simulink library "GridPackLib2"  (R2025b)
settings: Solver=VariableStepAuto  StartTime=0.0  StopTime=10.0  RelTol=1e-3
undefined symbols (not defined in the file): battery_builder_rtmsupport, gcbh
libraries: GridPackLib2_lib x2, nesl_utility x2
settings Model: Creator=User  LastModifiedBy=User

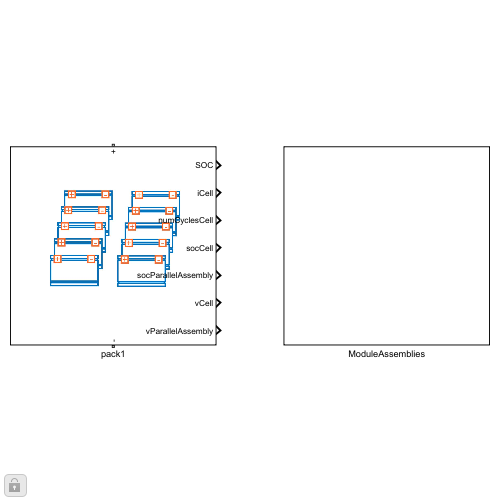
[thumbnail: Simulink's stored preview of the top-level diagram]
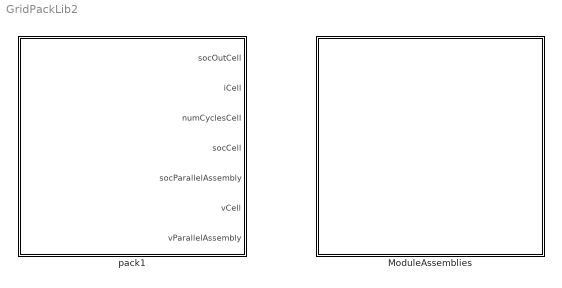
== system GridPackLib2 ==
  ModuleAssemblies : Subsystem
  pack1 : Subsystem  LoadFcn=battery_builder_rtmsupport('loadfcn',gcbh);
      settings: CopyFcn=battery_builder_rtmsupport('copyfcn',gcbh);  PreCopyFcn=battery_builder_rtmsupport('precopyfcn',gcbh);  PreDeleteFcn=battery_builder_rtmsupport('predeletefcn',gcbh);  PortSchema="{\"entries\":[{\"content\":{\"sides\":[{\"content\":{\"connectorIds\":[\"LConn1\"]},\"type\":\"ConnectorPlacement.EquallySpacedRectSide\",\"uuid\":\"88f5d390-8915-47fe-8d71-24cfaf6a6e27\"},{\"content\":{\"connectorIds\":[\"RConn1\"],\"side\":\"RIGHT\"},\"type\":\"ConnectorPlacement.EquallySpacedRectSide\",\"uuid\":\"89ebc1e9-5c7a-4e3e-b4ce-2bf86473cd1d\"},{\"content\":{\"side\":\"TOP\"},\"type\":\"ConnectorPlacement.EquallySpacedRectSide\",\"uuid\":\"3176116c-a81f-42a8-8903-646dc7856346\"},{\"content\":{\"connectorIds\":[\"Out1\",\"Out2\",\"Out3\",\"Out4\",\"Out5\",\"Out6\",\"Out7\"],\"side\":\"BOTTOM\"},\"type\":\"ConnectorPlacement.EquallySpacedRectSide\",\"uuid\":\"28216ba3-1a22-4e70-aa06-090b301a362d\"}]},\"type\":\"ConnectorPlacement.EquallySpacedConnector\",\"uuid\":\"25e0ce26-fb40-4ff1-8f8a-65e5050e8f25\"}],\"packageUris\":[\"http://schema.mathworks.com/mf0/Connector/R2020b\"],\"version\":\"1.0\"}"
      mask Display: image('$imagefile')

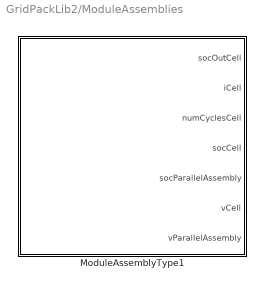
== system GridPackLib2/ModuleAssemblies ==
  ModuleAssemblyType1 : Subsystem  LoadFcn=battery_builder_rtmsupport('loadfcn',gcbh);
      settings: CopyFcn=battery_builder_rtmsupport('copyfcn',gcbh);  PreCopyFcn=battery_builder_rtmsupport('precopyfcn',gcbh);  PreDeleteFcn=battery_builder_rtmsupport('predeletefcn',gcbh);  PortSchema="{\"entries\":[{\"content\":{\"sides\":[{\"content\":{\"connectorIds\":[\"LConn1\"]},\"type\":\"ConnectorPlacement.EquallySpacedRectSide\",\"uuid\":\"88f5d390-8915-47fe-8d71-24cfaf6a6e27\"},{\"content\":{\"connectorIds\":[\"RConn1\"],\"side\":\"RIGHT\"},\"type\":\"ConnectorPlacement.EquallySpacedRectSide\",\"uuid\":\"89ebc1e9-5c7a-4e3e-b4ce-2bf86473cd1d\"},{\"content\":{\"side\":\"TOP\"},\"type\":\"ConnectorPlacement.EquallySpacedRectSide\",\"uuid\":\"3176116c-a81f-42a8-8903-646dc7856346\"},{\"content\":{\"connectorIds\":[\"Out1\",\"Out2\",\"Out3\",\"Out4\",\"Out5\",\"Out6\",\"Out7\"],\"side\":\"BOTTOM\"},\"type\":\"ConnectorPlacement.EquallySpacedRectSide\",\"uuid\":\"a9e7f8c6-f04c-4c1e-b058-680dc39e5ef0\"}]},\"type\":\"ConnectorPlacement.EquallySpacedConnector\",\"uuid\":\"25e0ce26-fb40-4ff1-8f8a-65e5050e8f25\"}],\"packageUris\":[\"http://schema.mathworks.com/mf0/Connector/R2020b\"],\"version\":\"1.0\"}"
      mask Display: image('$imagefile')

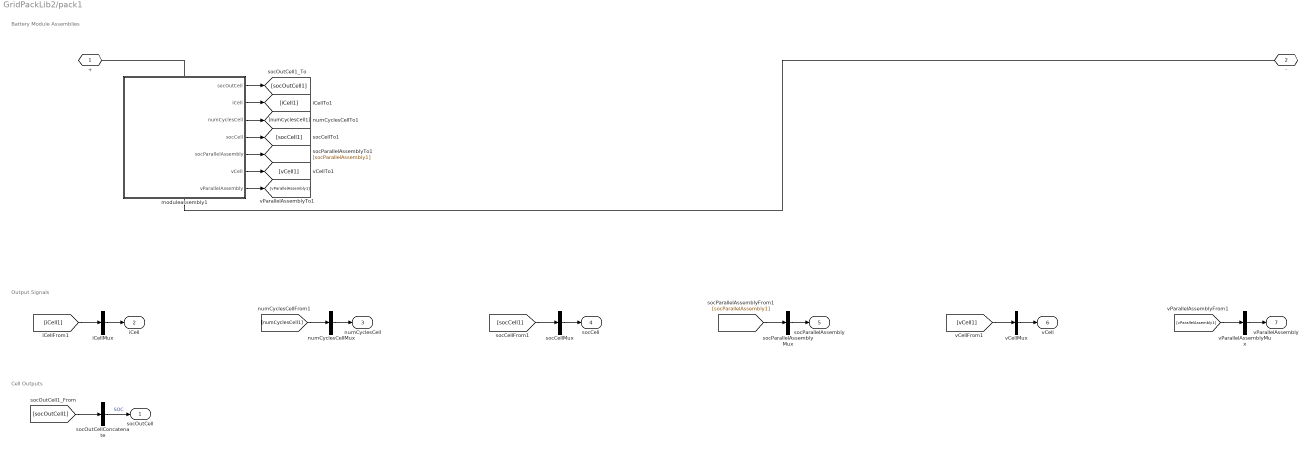
== system GridPackLib2/pack1 ==
  note: Battery Module Assemblies
  note: Output Signals
  note: Cell Outputs
  iCellMux : Mux  Inputs=1
  moduleassembly1 : Subsystem  LoadFcn=battery_builder_rtmsupport('loadfcn',gcbh);
      settings: CopyFcn=battery_builder_rtmsupport('copyfcn',gcbh);  PreCopyFcn=battery_builder_rtmsupport('precopyfcn',gcbh);  PreDeleteFcn=battery_builder_rtmsupport('predeletefcn',gcbh);  PortSchema="{\"entries\":[{\"content\":{\"sides\":[{\"content\":{\"connectorIds\":[\"LConn1\"]},\"type\":\"ConnectorPlacement.EquallySpacedRectSide\",\"uuid\":\"88f5d390-8915-47fe-8d71-24cfaf6a6e27\"},{\"content\":{\"connectorIds\":[\"RConn1\"],\"side\":\"RIGHT\"},\"type\":\"ConnectorPlacement.EquallySpacedRectSide\",\"uuid\":\"89ebc1e9-5c7a-4e3e-b4ce-2bf86473cd1d\"},{\"content\":{\"side\":\"TOP\"},\"type\":\"ConnectorPlacement.EquallySpacedRectSide\",\"uuid\":\"3176116c-a81f-42a8-8903-646dc7856346\"},{\"content\":{\"connectorIds\":[\"Out1\",\"Out2\",\"Out3\",\"Out4\",\"Out5\",\"Out6\",\"Out7\"],\"side\":\"BOTTOM\"},\"type\":\"ConnectorPlacement.EquallySpacedRectSide\",\"uuid\":\"a9e7f8c6-f04c-4c1e-b058-680dc39e5ef0\"}]},\"type\":\"ConnectorPlacement.EquallySpacedConnector\",\"uuid\":\"25e0ce26-fb40-4ff1-8f8a-65e5050e8f25\"}],\"packageUris\":[\"http://schema.mathworks.com/mf0/Connector/R2020b\"],\"version\":\"1.0\"}"
      mask Display: image('$imagefile')
  numCyclesCellMux : Mux  Inputs=1
  socCellMux : Mux  Inputs=1
  socOutCellConcatenate : Concatenate  NumInputs=1  Mode=Multidimensional array  ConcatenateDimension=2
  socParallelAssemblyMux : Mux  Inputs=1
  vCellMux : Mux  Inputs=1
  vParallelAssemblyMux : Mux  Inputs=1
  + : PMIOPort  Side=Left
  - : PMIOPort  Port=2  Side=Right
  socOutCell : Outport
  iCell : Outport  Port=2
  numCyclesCell : Outport  Port=3
  socCell : Outport  Port=4
  socParallelAssembly : Outport  Port=5
  vCell : Outport  Port=6
  vParallelAssembly : Outport  Port=7
  wires:
  socOutCellConcatenate/1 -> socOutCell/1  "SOC"
  [socOutCell1] -> socOutCellConcatenate/1
  moduleassembly1/2(iCell) -> [iCell1]
  iCellMux/1 -> iCell/1
  [iCell1] -> iCellMux/1
  moduleassembly1/3(numCyclesCell) -> [numCyclesCell1]
  numCyclesCellMux/1 -> numCyclesCell/1
  [numCyclesCell1] -> numCyclesCellMux/1
  moduleassembly1/4(socCell) -> [socCell1]
  socCellMux/1 -> socCell/1
  [socCell1] -> socCellMux/1
  moduleassembly1/5(socParallelAssembly) -> [socParallelAssembly1]
  socParallelAssemblyMux/1 -> socParallelAssembly/1
  [socParallelAssembly1] -> socParallelAssemblyMux/1
  moduleassembly1/6(vCell) -> [vCell1]
  vCellMux/1 -> vCell/1
  [vCell1] -> vCellMux/1
  moduleassembly1/7(vParallelAssembly) -> [vParallelAssembly1]
  vParallelAssemblyMux/1 -> vParallelAssembly/1
  [vParallelAssembly1] -> vParallelAssemblyMux/1
  moduleassembly1/1(socOutCell) -> [socOutCell1]
  connections:
  moduleassembly1/LConn1 -- +/RConn1
  moduleassembly1/RConn1 -- -/RConn1

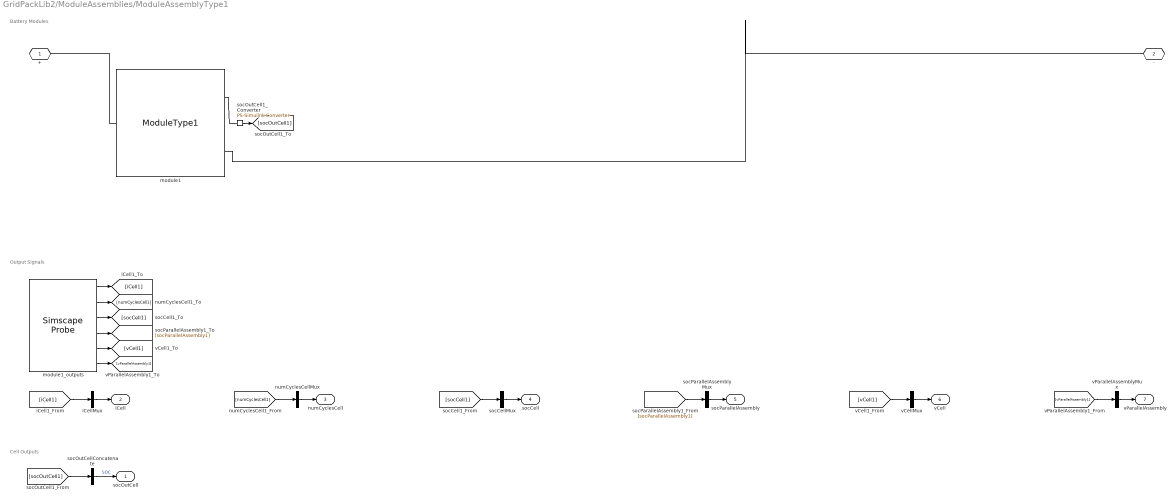
== system GridPackLib2/ModuleAssemblies/ModuleAssemblyType1 ==
  note: Battery Modules
  note: Output Signals
  note: Cell Outputs
  iCellMux : Mux  Inputs=1
  module1 : GridPackLib2_lib/Modules/ModuleType1  SOC_vecCell=[0, .01, .02, .03, .04, .05, .06, .07, .08, .09, .1, .11, .12, .13, .14, .15, .16, .17, .18, .19, .2, .21, .22, .23, .24, .25, .26, .27, .28, .29, .3, .31, .32, .33, .34, .35, .36, .37, .38, .39, .4, .41, .42, .43, .44, .45, .46, .47, .48, .49, .5, .51, .52, .53, .54, .55, .56, .57, .58, .59, .6, .61, .62, .63, .64, .65, .66, .67, .68, .69, .7, .71, .72, .73, .74, .75, .76, .77, .78, .79, .8, .81, .82, .83, .84, .85, .86, .87, .88, .89, .9, .91, .92, .93, .94, .95, .96, .97, .98, .99, 1]  V0_vecCell=[2.74087, 2.86425, 2.94379, 3.04526, 3.12652, 3.19558, 3.2527, 3.29775, 3.33159, 3.36, 3.3837, 3.4034, 3.41925, 3.43509, 3.4486, 3.45932, 3.47006, 3.47863, 3.48489, 3.49188, 3.49842, 3.50409, 3.50964, 3.51584, 3.52204, 3.52785, 3.53338, 3.53848, 3.54356, 3.54863, 3.55351, 3.55882, 3.56372, 3.56861, 3.5735, 3.57836, 3.58329, 3.58821, 3.59317, 3.59804, 3.60332, 3.60907, 3.61483, 3.62059, 3.62652, 3.6327, 3.63888, 3.64585, 3.65366, 3.66147, 3.66917, 3.67655, 3.68392, 3.69145, 3.69898, 3.70781, 3.71738, 3.72696, 3.73653, 3.74624, 3.75595, 3.7653, 3.77428, 3.7832, 3.79205, 3.8007, 3.80927, 3.8178, 3.82625, 3.83464, 3.84361, 3.85255, 3.86146, 3.87037, 3.87823, 3.88606, 3.89449, 3.90374, 3.91298, 3.9226, 3.93231, 3.94199, 3.95307, 3.96471, 3.97635, 3.98832, 4.00042, 4.01239, 4.02377, 4.03506, 4.04653, 4.05796, 4.06839, 4.07872, 4.08848, 4.09766, 4.10666, 4.11624, 4.12852, 4.14359, 4.22965] V  V_rangeCell=[2.475, Inf] V  R0_vecCell=[.3952, .44824, .45817, .49649, .51801, .52941, .53219, .52804, .51966, .50893, .49666, .48177, .46682, .45187, .43666, .42292, .40923, .39435, .37836, .3654, .35267, .33913, .32835, .31969, .31103, .30202, .29449, .28761, .28074, .27387, .26782, .26352, .25908, .25465, .2502, .2454, .24066, .23593, .23117, .22626, .22256, .22016, .21777, .21537, .21336, .21163, .20989, .20874, .20837, .208, .20731, .20564, .20397, .20226, .20055, .20026, .20086, .20147, .20207, .20264, .2032, .20269, .20183, .20093, .20005, .19903, .19783, .19654, .19527, .19397, .19325, .19243, .19151, .1906, .1887, .18671, .18502, .18504, .18507, .18543, .18518, .18483, .18547, .18641, .18735, .18945, .19195, .19411, .19486, .19553, .19661, .19791, .19879, .19998, .20083, .20074, .1989, .19723, .19215, .18252, .02326] Ohm  AHCell=0.716 A*hr  extrapolation_optionCell=simscape.enum.extrapolation.nearest  P=44  S=100  iCell_specify=off  iCell_priority=None  iCell=0 A  iCell_nominal_specify=off  iCell_nominal_value=1  iCell_nominal_unit=A  vCell_specify=off  vCell_priority=None  vCell=0 V  vCell_nominal_specify=off  vCell_nominal_value=1  vCell_nominal_unit=V  socCell_specify=off  socCell_priority=High  socCell=1  socCell_nominal_specify=off  socCell_nominal_value=1  socCell_nominal_unit=1  numCyclesCell_specify=off  numCyclesCell_priority=High  numCyclesCell=0  numCyclesCell_nominal_specify=off  numCyclesCell_nominal_value=1  numCyclesCell_nominal_unit=1  vParallelAssembly_specify=off  vParallelAssembly_priority=None  vParallelAssembly=repmat(0, 100, 1) V  vParallelAssembly_nominal_specify=off  vParallelAssembly_nominal_value=1  vParallelAssembly_nominal_unit=V  socParallelAssembly_specify=off  socParallelAssembly_priority=None  socParallelAssembly=repmat(1, 100, 1)  socParallelAssembly_nominal_specify=off  socParallelAssembly_nominal_value=1  socParallelAssembly_nominal_unit=1
      settings: InternalSimscapePortConfiguration="{\"Bottom\":[{\"id\":\"n\",\"label\":\"-\",\"type\":\"foundation.electrical.electrical\"}],\"Left\":[],\"Right\":[{\"id\":\"socOutCell\",\"label\":\"SOC\",\"type\":\"output\"}],\"Top\":[{\"id\":\"p\",\"label\":\"+\",\"type\":\"foundation.electrical.electrical\"}]}"
  module1_outputs : SimscapeProbe  BoundBlock=3  Variables="{\"iCell\":{\"Probing\":\"ON\"},\"numCyclesCell\":{\"Probing\":\"ON\"},\"socCell\":{\"Probing\":\"ON\"},\"socParallelAssembly\":{\"Probing\":\"ON\"},\"vCell\":{\"Probing\":\"ON\"},\"vParallelAssembly\":{\"Probing\":\"ON\"}}"
  numCyclesCellMux : Mux  Inputs=1
  socCellMux : Mux  Inputs=1
  socOutCell1_Converter : nesl_utility/PS-Simulink Converter  PhysicalDomain=network_engine_domain  SubClassName=ps_output  LeftPortType=input  RightPortType=output  PseudoPeriodic=off  Frequencies=[]  VectorFormat=inherit  Unit=inherit  AffineConversion=off
  socOutCellConcatenate : Concatenate  NumInputs=1  Mode=Multidimensional array  ConcatenateDimension=2
  socParallelAssemblyMux : Mux  Inputs=1
  vCellMux : Mux  Inputs=1
  vParallelAssemblyMux : Mux  Inputs=1
  + : PMIOPort  Side=Left
  - : PMIOPort  Port=2  Side=Right
  socOutCell : Outport
  iCell : Outport  Port=2
  numCyclesCell : Outport  Port=3
  socCell : Outport  Port=4
  socParallelAssembly : Outport  Port=5
  vCell : Outport  Port=6
  vParallelAssembly : Outport  Port=7
  wires:
  socOutCellConcatenate/1 -> socOutCell/1  "SOC"
  [socOutCell1] -> socOutCellConcatenate/1
  module1_outputs/1 -> [iCell1]
  iCellMux/1 -> iCell/1
  [iCell1] -> iCellMux/1
  module1_outputs/2 -> [numCyclesCell1]
  numCyclesCellMux/1 -> numCyclesCell/1
  [numCyclesCell1] -> numCyclesCellMux/1
  module1_outputs/3 -> [socCell1]
  socCellMux/1 -> socCell/1
  [socCell1] -> socCellMux/1
  module1_outputs/4 -> [socParallelAssembly1]
  socParallelAssemblyMux/1 -> socParallelAssembly/1
  [socParallelAssembly1] -> socParallelAssemblyMux/1
  module1_outputs/5 -> [vCell1]
  vCellMux/1 -> vCell/1
  [vCell1] -> vCellMux/1
  module1_outputs/6 -> [vParallelAssembly1]
  vParallelAssemblyMux/1 -> vParallelAssembly/1
  [vParallelAssembly1] -> vParallelAssemblyMux/1
  socOutCell1_Converter/1 -> [socOutCell1]
  connections:
  module1/LConn1 -- +/RConn1
  module1/RConn2 -- -/RConn1
  socOutCell1_Converter/LConn1 -- module1/RConn1

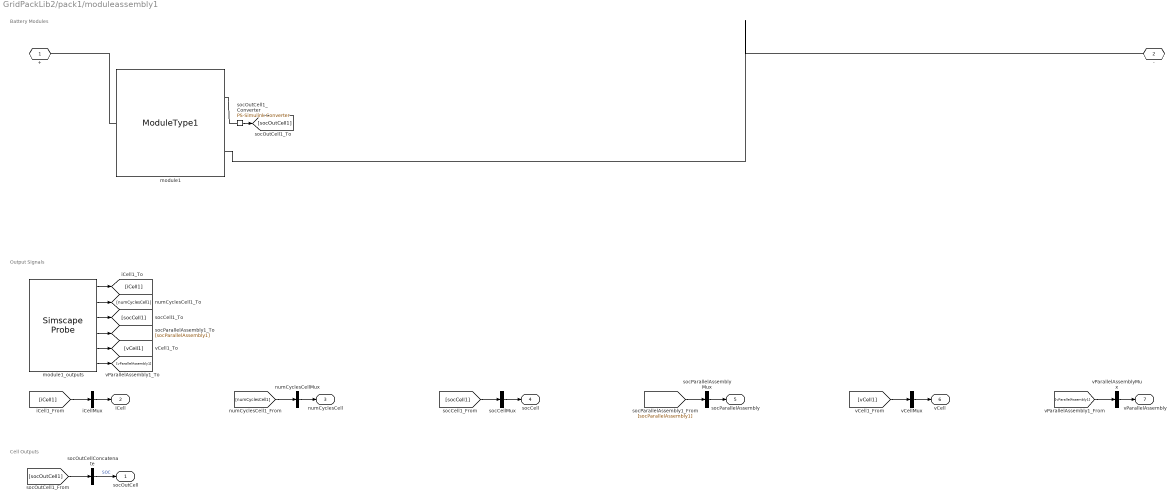
== system GridPackLib2/pack1/moduleassembly1 ==
  note: Cell Outputs
  note: Output Signals
  note: Battery Modules
  iCellMux : Mux  Inputs=1
  module1 : GridPackLib2_lib/Modules/ModuleType1  SOC_vecCell=[0, .01, .02, .03, .04, .05, .06, .07, .08, .09, .1, .11, .12, .13, .14, .15, .16, .17, .18, .19, .2, .21, .22, .23, .24, .25, .26, .27, .28, .29, .3, .31, .32, .33, .34, .35, .36, .37, .38, .39, .4, .41, .42, .43, .44, .45, .46, .47, .48, .49, .5, .51, .52, .53, .54, .55, .56, .57, .58, .59, .6, .61, .62, .63, .64, .65, .66, .67, .68, .69, .7, .71, .72, .73, .74, .75, .76, .77, .78, .79, .8, .81, .82, .83, .84, .85, .86, .87, .88, .89, .9, .91, .92, .93, .94, .95, .96, .97, .98, .99, 1]  V0_vecCell=[2.74087, 2.86425, 2.94379, 3.04526, 3.12652, 3.19558, 3.2527, 3.29775, 3.33159, 3.36, 3.3837, 3.4034, 3.41925, 3.43509, 3.4486, 3.45932, 3.47006, 3.47863, 3.48489, 3.49188, 3.49842, 3.50409, 3.50964, 3.51584, 3.52204, 3.52785, 3.53338, 3.53848, 3.54356, 3.54863, 3.55351, 3.55882, 3.56372, 3.56861, 3.5735, 3.57836, 3.58329, 3.58821, 3.59317, 3.59804, 3.60332, 3.60907, 3.61483, 3.62059, 3.62652, 3.6327, 3.63888, 3.64585, 3.65366, 3.66147, 3.66917, 3.67655, 3.68392, 3.69145, 3.69898, 3.70781, 3.71738, 3.72696, 3.73653, 3.74624, 3.75595, 3.7653, 3.77428, 3.7832, 3.79205, 3.8007, 3.80927, 3.8178, 3.82625, 3.83464, 3.84361, 3.85255, 3.86146, 3.87037, 3.87823, 3.88606, 3.89449, 3.90374, 3.91298, 3.9226, 3.93231, 3.94199, 3.95307, 3.96471, 3.97635, 3.98832, 4.00042, 4.01239, 4.02377, 4.03506, 4.04653, 4.05796, 4.06839, 4.07872, 4.08848, 4.09766, 4.10666, 4.11624, 4.12852, 4.14359, 4.22965] V  V_rangeCell=[2.475, Inf] V  R0_vecCell=[.3952, .44824, .45817, .49649, .51801, .52941, .53219, .52804, .51966, .50893, .49666, .48177, .46682, .45187, .43666, .42292, .40923, .39435, .37836, .3654, .35267, .33913, .32835, .31969, .31103, .30202, .29449, .28761, .28074, .27387, .26782, .26352, .25908, .25465, .2502, .2454, .24066, .23593, .23117, .22626, .22256, .22016, .21777, .21537, .21336, .21163, .20989, .20874, .20837, .208, .20731, .20564, .20397, .20226, .20055, .20026, .20086, .20147, .20207, .20264, .2032, .20269, .20183, .20093, .20005, .19903, .19783, .19654, .19527, .19397, .19325, .19243, .19151, .1906, .1887, .18671, .18502, .18504, .18507, .18543, .18518, .18483, .18547, .18641, .18735, .18945, .19195, .19411, .19486, .19553, .19661, .19791, .19879, .19998, .20083, .20074, .1989, .19723, .19215, .18252, .02326] Ohm  AHCell=0.716 A*hr  extrapolation_optionCell=simscape.enum.extrapolation.nearest  P=44  S=100  iCell_specify=off  iCell_priority=None  iCell=0 A  iCell_nominal_specify=off  iCell_nominal_value=1  iCell_nominal_unit=A  vCell_specify=off  vCell_priority=None  vCell=0 V  vCell_nominal_specify=off  vCell_nominal_value=1  vCell_nominal_unit=V  socCell_specify=off  socCell_priority=High  socCell=1  socCell_nominal_specify=off  socCell_nominal_value=1  socCell_nominal_unit=1  numCyclesCell_specify=off  numCyclesCell_priority=High  numCyclesCell=0  numCyclesCell_nominal_specify=off  numCyclesCell_nominal_value=1  numCyclesCell_nominal_unit=1  vParallelAssembly_specify=off  vParallelAssembly_priority=None  vParallelAssembly=repmat(0, 100, 1) V  vParallelAssembly_nominal_specify=off  vParallelAssembly_nominal_value=1  vParallelAssembly_nominal_unit=V  socParallelAssembly_specify=off  socParallelAssembly_priority=None  socParallelAssembly=repmat(1, 100, 1)  socParallelAssembly_nominal_specify=off  socParallelAssembly_nominal_value=1  socParallelAssembly_nominal_unit=1
      settings: InternalSimscapePortConfiguration="{\"Bottom\":[{\"id\":\"n\",\"label\":\"-\",\"type\":\"foundation.electrical.electrical\"}],\"Left\":[],\"Right\":[{\"id\":\"socOutCell\",\"label\":\"SOC\",\"type\":\"output\"}],\"Top\":[{\"id\":\"p\",\"label\":\"+\",\"type\":\"foundation.electrical.electrical\"}]}"
  module1_outputs : SimscapeProbe  BoundBlock=44  Variables="{\"iCell\":{\"Probing\":\"ON\"},\"numCyclesCell\":{\"Probing\":\"ON\"},\"socCell\":{\"Probing\":\"ON\"},\"socParallelAssembly\":{\"Probing\":\"ON\"},\"vCell\":{\"Probing\":\"ON\"},\"vParallelAssembly\":{\"Probing\":\"ON\"}}"
  numCyclesCellMux : Mux  Inputs=1
  socCellMux : Mux  Inputs=1
  socOutCell1_Converter : nesl_utility/PS-Simulink Converter  PhysicalDomain=network_engine_domain  SubClassName=ps_output  LeftPortType=input  RightPortType=output  PseudoPeriodic=off  Frequencies=[]  VectorFormat=inherit  Unit=inherit  AffineConversion=off
  socOutCellConcatenate : Concatenate  NumInputs=1  Mode=Multidimensional array  ConcatenateDimension=2
  socParallelAssemblyMux : Mux  Inputs=1
  vCellMux : Mux  Inputs=1
  vParallelAssemblyMux : Mux  Inputs=1
  + : PMIOPort  Side=Left
  - : PMIOPort  Port=2  Side=Right
  socOutCell : Outport
  iCell : Outport  Port=2
  numCyclesCell : Outport  Port=3
  socCell : Outport  Port=4
  socParallelAssembly : Outport  Port=5
  vCell : Outport  Port=6
  vParallelAssembly : Outport  Port=7
  wires:
  socOutCell1_Converter/1 -> [socOutCell1]
  [vParallelAssembly1] -> vParallelAssemblyMux/1
  vParallelAssemblyMux/1 -> vParallelAssembly/1
  module1_outputs/6 -> [vParallelAssembly1]
  [vCell1] -> vCellMux/1
  vCellMux/1 -> vCell/1
  module1_outputs/5 -> [vCell1]
  [socParallelAssembly1] -> socParallelAssemblyMux/1
  socParallelAssemblyMux/1 -> socParallelAssembly/1
  module1_outputs/4 -> [socParallelAssembly1]
  [socCell1] -> socCellMux/1
  socCellMux/1 -> socCell/1
  module1_outputs/3 -> [socCell1]
  [numCyclesCell1] -> numCyclesCellMux/1
  numCyclesCellMux/1 -> numCyclesCell/1
  module1_outputs/2 -> [numCyclesCell1]
  [iCell1] -> iCellMux/1
  iCellMux/1 -> iCell/1
  module1_outputs/1 -> [iCell1]
  [socOutCell1] -> socOutCellConcatenate/1
  socOutCellConcatenate/1 -> socOutCell/1  "SOC"
  connections:
  socOutCell1_Converter/LConn1 -- module1/RConn1
  module1/RConn2 -- -/RConn1
  module1/LConn1 -- +/RConn1
